simulink model "GHAME_Trim"  (R2024a)
settings: Solver=ode4  StartTime=0.0  StopTime=30  FixedStep=0.01  RelTol=1e-3
undefined symbols (not defined in the file): Data, IC, Sim
libraries: simulink_extras x4, sharedutil x2
settings Model: PauseTimes=399.98  PacingRate=1000  Creator=Thoma  LastModifiedBy=muel_td
settings SolverCC: AlgebraicLoopSolver=TrustRegion
settings DataIOCC: ExternalInput=getinputstruct(report2)  InitialState=getstatestruct(report2)
settings DebuggingCC: AlgebraicLoopMsg=none  InitInArrayFormatMsg=none  ArithmeticOperatorsInVariantConditions=warning
settings SFSimCC: CustomCodeUndefinedFunction=UseInterfaceOnly
settings RTWCC: GPUComputeCapability=3.5

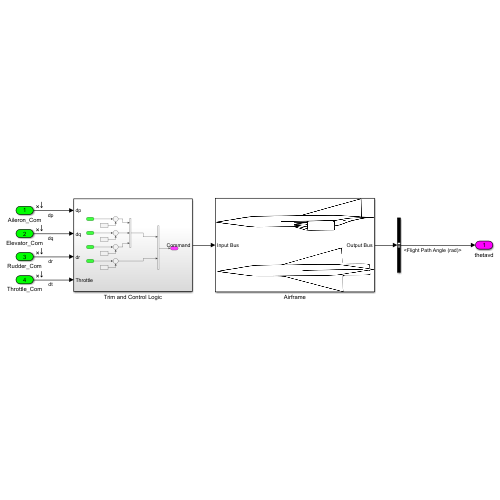
[thumbnail: Simulink's stored preview of the top-level diagram]
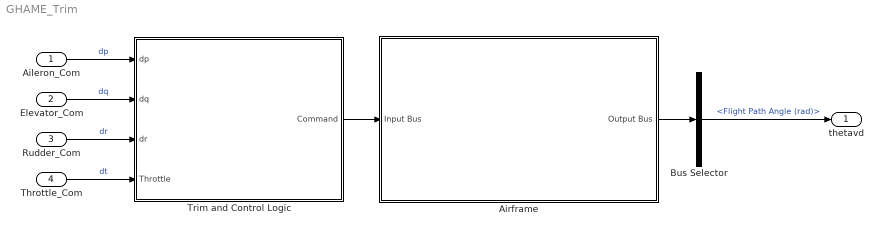
== system GHAME_Trim ==
  Aileron_Com : Inport  OutDataTypeStr=double
  Elevator_Com : Inport  Port=2  OutDataTypeStr=double
  Rudder_Com : Inport  Port=3  OutDataTypeStr=double
  Throttle_Com : Inport  Port=4
  Airframe : Subsystem
      mask Display: image('GHAME.png'); % Use "Edit Image" on toolstrip to change.
  Bus Selector : BusSelector  OutputSignals=Flight Path Angle (rad)
  Trim and Control Logic : Subsystem
  thetavd : Outport
  wires:
  Airframe/1(Output Bus) -> Bus Selector/1
  Bus Selector/1 -> thetavd/1  "<Flight Path Angle (rad)>"
  Aileron_Com/1 -> Trim and Control Logic/1(dp)  "dp"
  Elevator_Com/1 -> Trim and Control Logic/2(dq)  "dq"
  Rudder_Com/1 -> Trim and Control Logic/3(dr)  "dr"
  Throttle_Com/1 -> Trim and Control Logic/4(Throttle)  "dt"
  Trim and Control Logic/1(Command) -> Airframe/1(Input Bus)

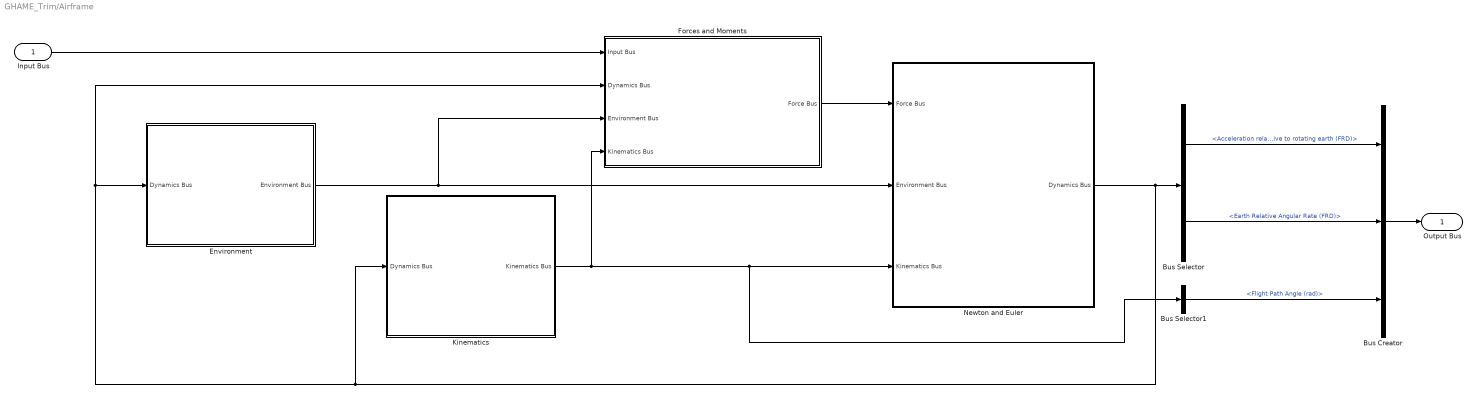
== system GHAME_Trim/Airframe ==
  Input Bus : Inport
  Bus Creator : BusCreator  Inputs=3
  Bus Selector : BusSelector  OutputSignals=Acceleration relative to rotating earth (FRD),Earth Relative Angular Rate (FRD)
  Bus Selector1 : BusSelector  OutputSignals=Flight Path Angle (rad)
  Environment : Subsystem
  Forces and Moments : Subsystem
  Kinematics : Subsystem
  Newton and Euler : Subsystem
  Output Bus : Outport
  wires:
  Newton and Euler/1(Dynamics Bus) -> Forces and Moments/2(Dynamics Bus), Environment/1(Dynamics Bus), Kinematics/1(Dynamics Bus), Bus Selector/1
  Kinematics/1(Kinematics Bus) -> Bus Selector1/1, Newton and Euler/3(Kinematics Bus), Forces and Moments/4(Kinematics Bus)
  Environment/1(Environment Bus) -> Forces and Moments/3(Environment Bus), Newton and Euler/2(Environment Bus)
  Forces and Moments/1(Force Bus) -> Newton and Euler/1(Force Bus)
  Input Bus/1 -> Forces and Moments/1(Input Bus)
  Bus Creator/1 -> Output Bus/1
  Bus Selector1/1 -> Bus Creator/3  "<Flight Path Angle (rad)>"
  Bus Selector/2 -> Bus Creator/2  "<Earth Relative Angular Rate (FRD)>"
  Bus Selector/1 -> Bus Creator/1  "<Acceleration relative to rotating earth (FRD)>"

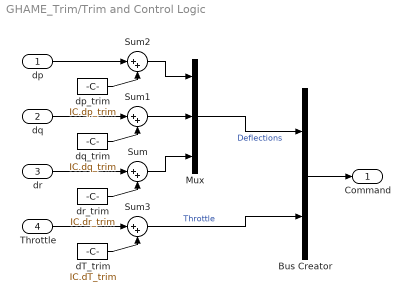
== system GHAME_Trim/Trim and Control Logic ==
  dp : Inport
  dq : Inport  Port=2
  dr : Inport  Port=3
  Throttle : Inport  Port=4
  Bus Creator : BusCreator  Inputs=2
  Mux : Mux  Inputs=3
  Sum{,1..3} (4 alike) : Sum  Inputs=|++
  dT_trim : Constant  Value=IC.dT_trim
  dp_trim : Constant  Value=IC.dp_trim
  dq_trim : Constant  Value=IC.dq_trim
  dr_trim : Constant  Value=IC.dr_trim
  Command : Outport
  wires:
  dr_trim/1 -> Sum/2
  Mux/1 -> Bus Creator/1  "Deflections"
  dq_trim/1 -> Sum1/2
  dp_trim/1 -> Sum2/2
  Sum/1 -> Mux/3
  Sum2/1 -> Mux/1
  Sum1/1 -> Mux/2
  dT_trim/1 -> Sum3/2
  Sum3/1 -> Bus Creator/2  "Throttle"
  Bus Creator/1 -> Command/1
  Throttle/1 -> Sum3/1
  dr/1 -> Sum/1
  dq/1 -> Sum1/1
  dp/1 -> Sum2/1

== system GHAME_Trim/Airframe/Environment ==
  Dynamics Bus : Inport
  Bus Creator : BusCreator  Inputs=5
  Bus Selector : BusSelector  OutputSignals=Geographic Velocity [NED],Geodetic Altitude,Inertial Position
  ENVIRONMENT : Subsystem
  Environment Bus : Outport
  wires:
  ENVIRONMENT/2(rho) -> Bus Creator/2  "Air Density"
  ENVIRONMENT/1(GRAVG) -> Bus Creator/1  "Gravitation (NED)"
  ENVIRONMENT/3(pdynmc) -> Bus Creator/3  "Dynamic Pressure"
  ENVIRONMENT/5(dvba) -> Bus Creator/5  "True Airspeed"
  ENVIRONMENT/4(vmach) -> Bus Creator/4  "Mach Number"
  Bus Creator/1 -> Environment Bus/1
  Dynamics Bus/1 -> Bus Selector/1
  Bus Selector/1 -> ENVIRONMENT/1(VBED)  "<Geographic Velocity [NED]>"
  Bus Selector/3 -> ENVIRONMENT/3(SBII)  "<Inertial Position>"
  Bus Selector/2 -> ENVIRONMENT/2(alt)  "<Geodetic Altitude>"

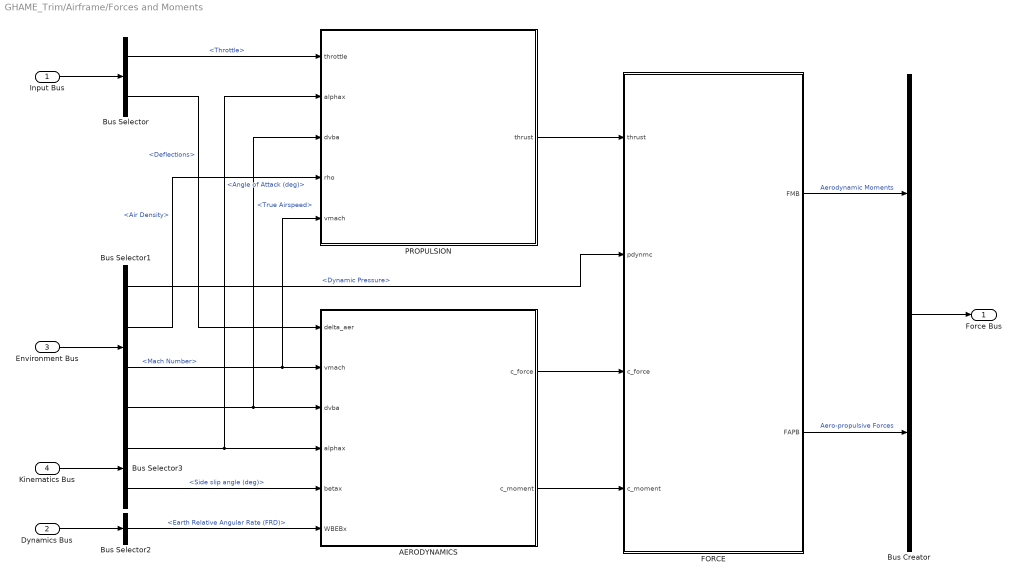
== system GHAME_Trim/Airframe/Forces and Moments ==
  Input Bus : Inport
  Dynamics Bus : Inport  Port=2
  Environment Bus : Inport  Port=3
  Kinematics Bus : Inport  Port=4
  AERODYNAMICS : Subsystem
  Bus Creator : BusCreator  Inputs=2
  Bus Selector : BusSelector  OutputSignals=Throttle,Deflections
  Bus Selector1 : BusSelector  OutputSignals=Dynamic Pressure,Air Density,Mach Number,True Airspeed
  Bus Selector2 : BusSelector  OutputSignals=Earth Relative Angular Rate (FRD)
  Bus Selector3 : BusSelector  OutputSignals=Angle of Attack (deg),Side slip angle (deg)
  FORCE : Subsystem
  PROPULSION : Subsystem
  Force Bus : Outport
  wires:
  Input Bus/1 -> Bus Selector/1
  Environment Bus/1 -> Bus Selector1/1
  Bus Selector/1 -> PROPULSION/1(throttle)  "<Throttle>"
  PROPULSION/1(thrust) -> FORCE/1(thrust)
  AERODYNAMICS/1(c_force) -> FORCE/3(c_force)
  AERODYNAMICS/2(c_moment) -> FORCE/4(c_moment)
  Bus Selector1/3 -> PROPULSION/5(vmach), AERODYNAMICS/2(vmach)  "<Mach Number>"
  Bus Selector1/4 -> PROPULSION/3(dvba), AERODYNAMICS/3(dvba)  "<True Airspeed>"
  Bus Selector1/2 -> PROPULSION/4(rho)  "<Air Density>"
  Dynamics Bus/1 -> Bus Selector2/1
  Bus Selector2/1 -> AERODYNAMICS/6(WBEBx)  "<Earth Relative Angular Rate (FRD)>"
  Kinematics Bus/1 -> Bus Selector3/1
  Bus Selector3/1 -> AERODYNAMICS/4(alphax), PROPULSION/2(alphax)  "<Angle of Attack (deg)>"
  Bus Selector3/2 -> AERODYNAMICS/5(betax)  "<Side slip angle (deg)>"
  FORCE/1(FMB) -> Bus Creator/1  "Aerodynamic Moments"
  FORCE/2(FAPB) -> Bus Creator/2  "Aero-propulsive Forces"
  Bus Creator/1 -> Force Bus/1
  Bus Selector/2 -> AERODYNAMICS/1(delta_aer)  "<Deflections>"
  Bus Selector1/1 -> FORCE/2(pdynmc)  "<Dynamic Pressure>"

== system GHAME_Trim/Airframe/Kinematics ==
  Dynamics Bus : Inport
  Bus Creator : BusCreator  Inputs=7
  Bus Selector : BusSelector  OutputSignals=Acceleration relative to rotating earth (FRD),Earth Relative Angular Rate (FRD),Geographic Velocity [NED],Inertial to Geodetic TM
  KINEMATICS : Subsystem
  Kinematics Bus : Outport
  wires:
  Dynamics Bus/1 -> Bus Selector/1
  Bus Selector/3 -> KINEMATICS/3(VBED)  "<Geographic Velocity [NED]>"
  Bus Selector/2 -> KINEMATICS/2(WBEBx)  "<Earth Relative Angular Rate (FRD)>"
  Bus Selector/1 -> KINEMATICS/1(a_BE_B)  "<Acceleration relative to rotating earth (FRD)>"
  KINEMATICS/1(e_BD) -> Bus Creator/1  "Euler Angles (rad)"
  KINEMATICS/2(TBD) -> Bus Creator/2  "Geodetic to Body TM"
  KINEMATICS/3(alphax) -> Bus Creator/3  "Angle of Attack (deg)"
  KINEMATICS/4(betax) -> Bus Creator/4  "Side slip angle (deg)"
  KINEMATICS/5(VBAB) -> Bus Creator/5  "Aerodynamic Velocity (FRD)"
  KINEMATICS/6(TBI) -> Bus Creator/6  "Inertial to Body TM"
  Bus Creator/1 -> Kinematics Bus/1
  Bus Selector/4 -> KINEMATICS/4(TDI)  "<Inertial to Geodetic TM>"
  KINEMATICS/7(thetavd) -> Bus Creator/7  "Flight Path Angle (rad)"

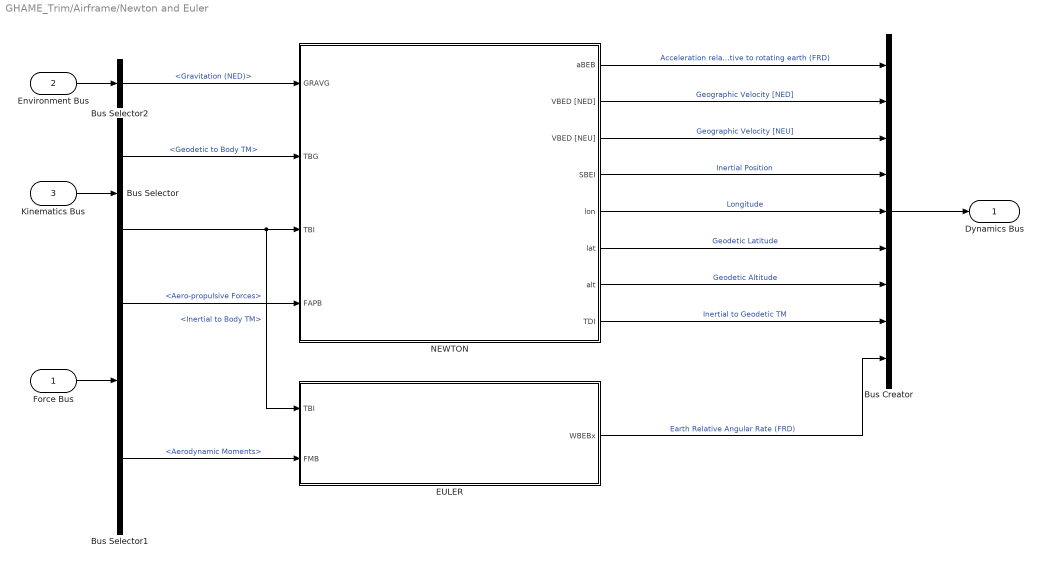
== system GHAME_Trim/Airframe/Newton and Euler ==
  Force Bus : Inport
  Environment Bus : Inport  Port=2
  Kinematics Bus : Inport  Port=3
  Bus Creator : BusCreator  Inputs=9
  Bus Selector : BusSelector  OutputSignals=Geodetic to Body TM,Inertial to Body TM
  Bus Selector1 : BusSelector  OutputSignals=Aero-propulsive Forces,Aerodynamic Moments
  Bus Selector2 : BusSelector  OutputSignals=Gravitation (NED)
  EULER : Subsystem
  NEWTON : Subsystem
  Dynamics Bus : Outport
  wires:
  Bus Selector1/2 -> EULER/2(FMB)  "<Aerodynamic Moments>"
  Bus Selector1/1 -> NEWTON/4(FAPB)  "<Aero-propulsive Forces>"
  Bus Creator/1 -> Dynamics Bus/1
  NEWTON/1(aBEB) -> Bus Creator/1  "Acceleration relative to rotating earth (FRD)"
  NEWTON/2(VBED [NED]) -> Bus Creator/2  "Geographic Velocity [NED]"
  NEWTON/3(VBED [NEU]) -> Bus Creator/3  "Geographic Velocity [NEU]"
  NEWTON/4("SBEI ") -> Bus Creator/4  "Inertial Position"
  NEWTON/5(lon) -> Bus Creator/5  "Longitude"
  NEWTON/6(lat) -> Bus Creator/6  "Geodetic Latitude"
  NEWTON/7(alt) -> Bus Creator/7  "Geodetic Altitude"
  Kinematics Bus/1 -> Bus Selector/1
  Bus Selector/2 -> NEWTON/3(TBI), EULER/1(TBI)  "<Inertial to Body TM>"
  Force Bus/1 -> Bus Selector1/1
  Bus Selector/1 -> NEWTON/2(TBG)  "<Geodetic to Body TM>"
  Environment Bus/1 -> Bus Selector2/1
  Bus Selector2/1 -> NEWTON/1(GRAVG)  "<Gravitation (NED)>"
  NEWTON/8(TDI) -> Bus Creator/8  "Inertial to Geodetic TM"
  EULER/1(WBEBx) -> Bus Creator/9  "Earth Relative Angular Rate (FRD)"

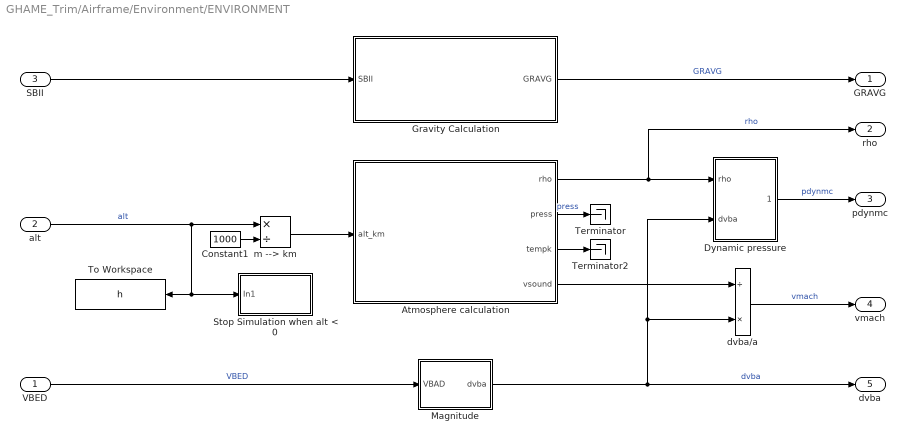
== system GHAME_Trim/Airframe/Environment/ENVIRONMENT ==
  VBED : Inport
  alt : Inport  Port=2
  SBII : Inport  Port=3
  Atmosphere calculation : MATLAB Function  Priority=2  TreatAsAtomicUnit=on
  Constant1 : Constant  Value=1000
  Dynamic pressure : Subsystem
  Gravity Calculation : MATLAB Function  Priority=1  TreatAsAtomicUnit=on
  Magnitude : MATLAB Function  TreatAsAtomicUnit=on
  Stop Simulation when alt < 0 : Subsystem
  Terminator : Terminator
  Terminator2 : Terminator
  To Workspace : ToWorkspace  VariableName=h  SampleTime=-1
  dvba/a : Product  Inputs=/*
  m --> km : Product  Inputs=*/
  GRAVG : Outport
  rho : Outport  Port=2
  pdynmc : Outport  Port=3
  vmach : Outport  Port=4
  dvba : Outport  Port=5
  wires:
  alt/1 -> To Workspace/1, Stop Simulation when alt < 0/1(In1), m --> km/1  "alt"
  Atmosphere calculation/3(tempk) -> Terminator2/1
  Constant1/1 -> m --> km/2
  m --> km/1 -> Atmosphere calculation/1(alt_km)
  dvba/a/1 -> vmach/1  "vmach"
  Atmosphere calculation/1(rho) -> Dynamic pressure/1(rho), rho/1  "rho"
  Dynamic pressure/1(pdynmc) -> pdynmc/1  "pdynmc"
  Atmosphere calculation/4(vsound) -> dvba/a/1
  Magnitude/1(dvba) -> dvba/a/2, Dynamic pressure/2(dvba), dvba/1  "dvba"
  Gravity Calculation/1(GRAVG) -> GRAVG/1  "GRAVG"
  SBII/1 -> Gravity Calculation/1(SBII)
  VBED/1 -> Magnitude/1(VBAD)  "VBED"
  Atmosphere calculation/2(press) -> Terminator/1  "press"

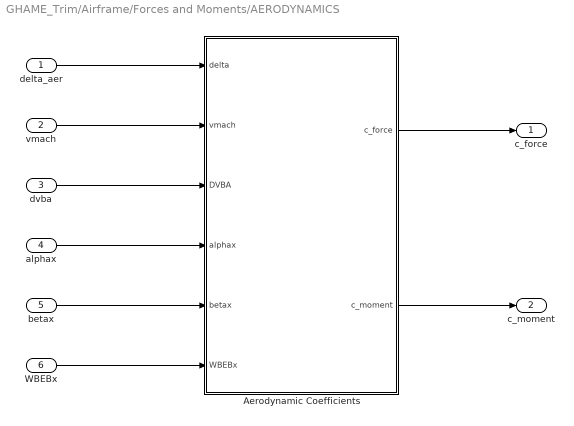
== system GHAME_Trim/Airframe/Forces and Moments/AERODYNAMICS ==
  delta_aer : Inport
  vmach : Inport  Port=2
  dvba : Inport  Port=3
  alphax : Inport  Port=4
  betax : Inport  Port=5
  WBEBx : Inport  Port=6
  Aerodynamic Coefficients : MATLAB Function  TreatAsAtomicUnit=on
  c_force : Outport  PortDimensions=[3 1]
  c_moment : Outport  Port=2  PortDimensions=[3 1]
  wires:
  vmach/1 -> Aerodynamic Coefficients/2(vmach)
  dvba/1 -> Aerodynamic Coefficients/3(DVBA)
  betax/1 -> Aerodynamic Coefficients/5(betax)
  alphax/1 -> Aerodynamic Coefficients/4(alphax)
  Aerodynamic Coefficients/1(c_force) -> c_force/1
  WBEBx/1 -> Aerodynamic Coefficients/6(WBEBx)
  Aerodynamic Coefficients/2(c_moment) -> c_moment/1
  delta_aer/1 -> Aerodynamic Coefficients/1(delta)

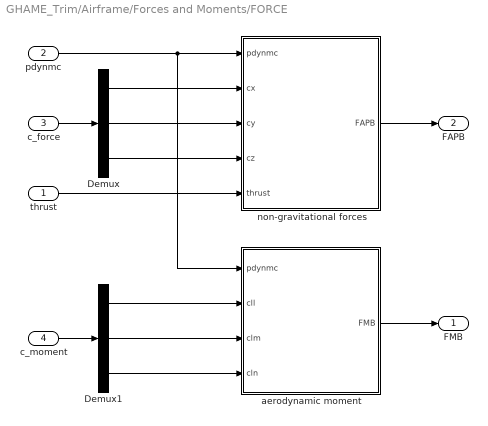
== system GHAME_Trim/Airframe/Forces and Moments/FORCE ==
  thrust : Inport
  pdynmc : Inport  Port=2
  c_force : Inport  Port=3  PortDimensions=[3 1]
  c_moment : Inport  Port=4  PortDimensions=[3 1]
  Demux : Demux  Outputs=3
  Demux1 : Demux  Outputs=3
  aerodynamic moment : MATLAB Function  TreatAsAtomicUnit=on
  non-gravitational forces : MATLAB Function  TreatAsAtomicUnit=on
  FMB : Outport
  FAPB : Outport  Port=2
  wires:
  Demux/1 -> non-gravitational forces/2(cx)
  c_force/1 -> Demux/1
  Demux/3 -> non-gravitational forces/4(cz)
  non-gravitational forces/1(FAPB) -> FAPB/1
  Demux1/1 -> aerodynamic moment/2(cll)
  c_moment/1 -> Demux1/1
  Demux1/3 -> aerodynamic moment/4(cln)
  aerodynamic moment/1(FMB) -> FMB/1
  Demux/2 -> non-gravitational forces/3(cy)
  Demux1/2 -> aerodynamic moment/3(clm)
  thrust/1 -> non-gravitational forces/5(thrust)
  pdynmc/1 -> non-gravitational forces/1(pdynmc), aerodynamic moment/1(pdynmc)

== system GHAME_Trim/Airframe/Forces and Moments/PROPULSION ==
  throttle : Inport
  alphax : Inport  Port=2
  dvba : Inport  Port=3
  rho : Inport  Port=4
  vmach : Inport  Port=5
  making thrust calculations : MATLAB Function  TreatAsAtomicUnit=on
  thrust : Outport
  wires:
  rho/1 -> making thrust calculations/1(rho)
  dvba/1 -> making thrust calculations/4(DVBA)
  vmach/1 -> making thrust calculations/2(Mach)
  making thrust calculations/1(Thrust) -> thrust/1  "Thrust"
  alphax/1 -> making thrust calculations/3(alphax)
  throttle/1 -> making thrust calculations/5(Throttle)

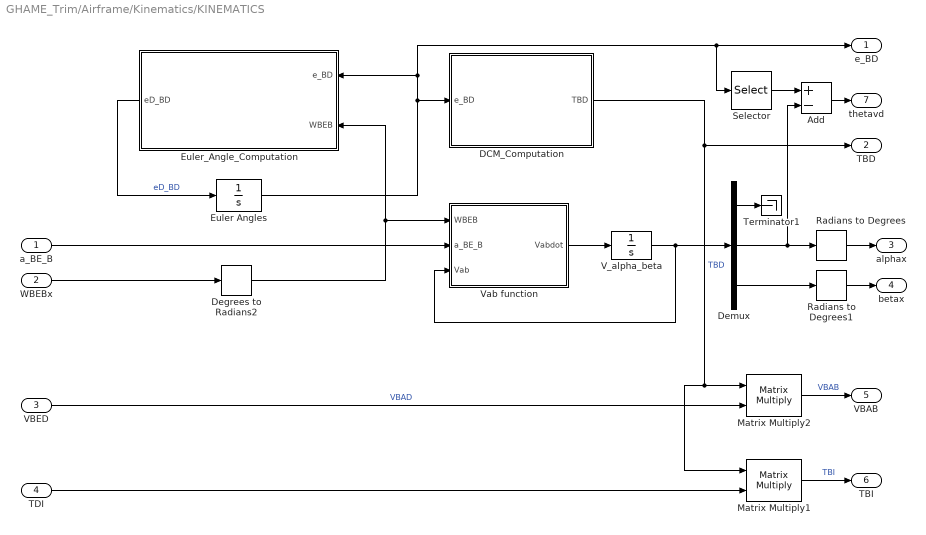
== system GHAME_Trim/Airframe/Kinematics/KINEMATICS ==
  a_BE_B : Inport
  WBEBx : Inport  Port=2
  VBED : Inport  Port=3
  TDI : Inport  Port=4
  Add : Sum  Inputs=+-
  DCM_Computation : MATLAB Function  TreatAsAtomicUnit=on
  Degrees to Radians2 : simulink_extras/Transformations/Degrees to Radians
  Demux : Demux  Outputs=3
  Euler Angles : Integrator  InitialCondition=[IC.psibd; IC.thtbd; IC.phibd]
  Euler_Angle_Computation : MATLAB Function  TreatAsAtomicUnit=on
  Matrix Multiply1 : Product  Multiplication=Matrix(*)
  Matrix Multiply2 : Product  Multiplication=Matrix(*)
  Radians to Degrees : simulink_extras/Transformations/Radians to Degrees
  Radians to Degrees1 : simulink_extras/Transformations/Radians to Degrees
  Selector : Selector  InputPortWidth=3  IndexOptions=Index vector (dialog)  Indices=[2]  OutputSizes=1
  Terminator1 : Terminator
  V_alpha_beta : Integrator  InitialCondition=[IC.dvba; IC.alpha; 0]
  Vab function : MATLAB Function  TreatAsAtomicUnit=on
  e_BD : Outport
  TBD : Outport  Port=2
  alphax : Outport  Port=3
  betax : Outport  Port=4
  VBAB : Outport  Port=5
  TBI : Outport  Port=6
  thetavd : Outport  Port=7
  wires:
  Matrix Multiply1/1 -> TBI/1  "TBI"
  VBED/1 -> Matrix Multiply2/2  "VBAD"
  WBEBx/1 -> Degrees to Radians2/1
  Euler Angles/1 -> e_BD/1, Selector/1, Euler_Angle_Computation/1(e_BD), DCM_Computation/1(e_BD)
  DCM_Computation/1(TBD) -> TBD/1, Matrix Multiply1/1, Matrix Multiply2/1  "TBD"
  Euler_Angle_Computation/1(eD_BD) -> Euler Angles/1  "eD_BD"
  Vab function/1(Vabdot) -> V_alpha_beta/1
  V_alpha_beta/1 -> Vab function/3(Vab), Demux/1
  Demux/1 -> Terminator1/1
  Demux/3 -> Radians to Degrees1/1
  a_BE_B/1 -> Vab function/2(a_BE_B)
  Degrees to Radians2/1 -> Euler_Angle_Computation/2(WBEB), Vab function/1(WBEB)
  Demux/2 -> Radians to Degrees/1, Add/2
  Matrix Multiply2/1 -> VBAB/1  "VBAB"
  TDI/1 -> Matrix Multiply1/2
  Selector/1 -> Add/1
  Add/1 -> thetavd/1
  Radians to Degrees/1 -> alphax/1
  Radians to Degrees1/1 -> betax/1

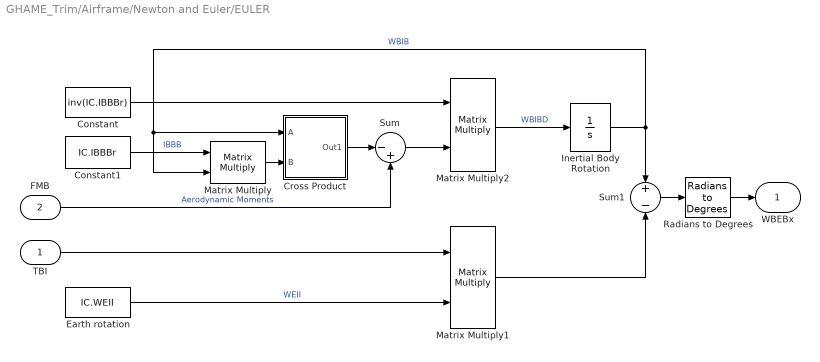
== system GHAME_Trim/Airframe/Newton and Euler/EULER ==
  TBI : Inport
  FMB : Inport  Port=2
  Constant : Constant  Value=inv(IC.IBBBr)
  Constant1 : Constant  Value=IC.IBBBr
  Cross Product : Subsystem
  Earth rotation : Constant  Value=IC.WEII
  Inertial Body Rotation : Integrator  InitialCondition=IC.WBIB
  Matrix Multiply : Product  Multiplication=Matrix(*)
  Matrix Multiply1 : Product  Multiplication=Matrix(*)
  Matrix Multiply2 : Product  Multiplication=Matrix(*)
  Radians to Degrees : simulink_extras/Transformations/Radians to Degrees
  Sum : Sum  Inputs=|-+
  Sum1 : Sum  Inputs=+-
  WBEBx : Outport
  wires:
  FMB/1 -> Sum/2  "Aerodynamic Moments"
  Matrix Multiply2/1 -> Inertial Body Rotation/1  "WBIBD"
  Constant1/1 -> Matrix Multiply/1  "IBBB"
  Inertial Body Rotation/1 -> Sum1/1, Cross Product/1(A), Matrix Multiply/2  "WBIB"
  Matrix Multiply/1 -> Cross Product/2(B)
  Sum/1 -> Matrix Multiply2/2
  Radians to Degrees/1 -> WBEBx/1
  Cross Product/1(Out1) -> Sum/1
  Constant/1 -> Matrix Multiply2/1
  TBI/1 -> Matrix Multiply1/1
  Earth rotation/1 -> Matrix Multiply1/2  "WEII"
  Matrix Multiply1/1 -> Sum1/2
  Sum1/1 -> Radians to Degrees/1

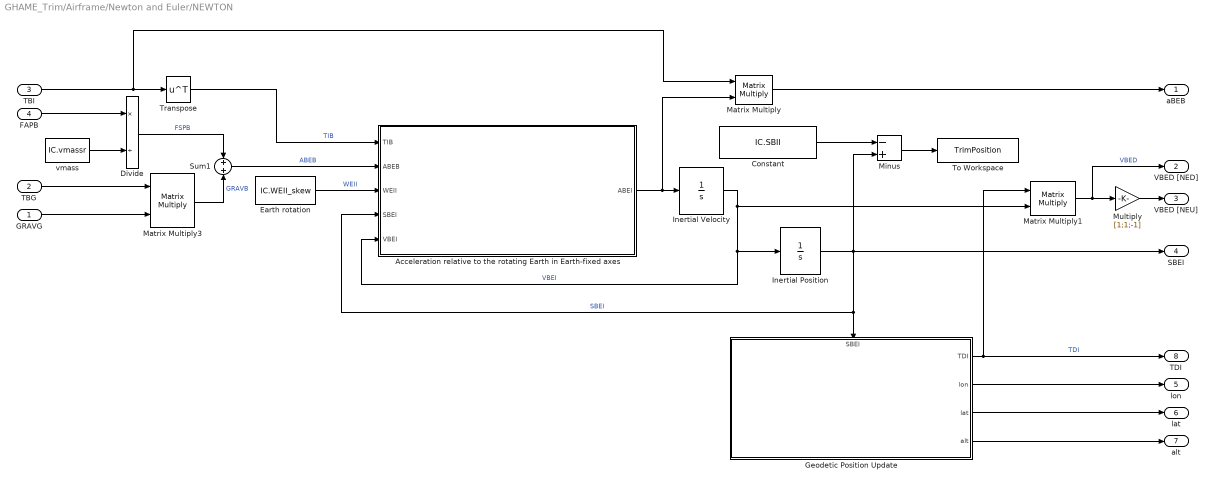
== system GHAME_Trim/Airframe/Newton and Euler/NEWTON ==
  GRAVG : Inport
  TBG : Inport  Port=2
  TBI : Inport  Port=3
  FAPB : Inport  Port=4
  Acceleration relative to the rotating Earth in Earth-fixed axes : Subsystem
  Constant : Constant  Value=IC.SBII  SampleTime=Sim.sample_time
  Divide : Product  Inputs=*/
  Earth rotation : Constant  Value=IC.WEII_skew
  Geodetic Position Update : Subsystem
      settings: PortSchema="{\"entries\":[{\"content\":{\"sides\":[{\"content\":{},\"type\":\"ConnectorPlacement.EquallySpacedRectSide\",\"uuid\":\"95933ad7-71e7-41f9-a46f-bd289a95730a\"},{\"content\":{\"connectorIds\":[\"Out1\",\"Out2\",\"Out3\",\"Out4\"],\"side\":\"RIGHT\"},\"type\":\"ConnectorPlacement.EquallySpacedRectSide\",\"uuid\":\"ab2689fc-78b4-4a63-be7d-36d19ac80c5e\"},{\"content\":{\"connectorIds\":[\"In1\"],\"side\":\"TOP\"},\"type\":\"ConnectorPlacement.EquallySpacedRectSide\",\"uuid\":\"1c090c4e-beeb-4e17-b6f2-47983e28fdde\"}]},\"type\":\"ConnectorPlacement.EquallySpacedConnector\",\"uuid\":\"92176c65-9b1a-45aa-814d-7bd7a5ccaffc\"}],\"packageUris\":[\"http://schema.mathworks.com/mf0/Connector/R2020b\"],\"version\":\"1.0\"}"
  Inertial Position : Integrator  InitialCondition=IC.SBII
  Inertial Velocity : Integrator  InitialCondition=IC.VBEI
  Matrix Multiply : Product  Multiplication=Matrix(*)
  Matrix Multiply1 : Product  Multiplication=Matrix(*)
  Matrix Multiply3 : Product  Multiplication=Matrix(*)
  Minus : Sum  Inputs=-+
  Multiply : Gain  Gain=[1;1;-1]
  Sum1 : Sum
  To Workspace : ToWorkspace  VariableName=TrimPosition  SaveFormat=Timeseries  SampleTime=-1
  Transpose : Math  Operator=transpose  SignedPower=on
  vmass : Constant  Value=IC.vmassr
  aBEB : Outport
  VBED [NED] : Outport  Port=2
  VBED [NEU] : Outport  Port=3
  "SBEI " : Outport  Port=4
  lon : Outport  Port=5
  lat : Outport  Port=6
  alt : Outport  Port=7
  TDI : Outport  Port=8
  wires:
  TBG/1 -> Matrix Multiply3/1
  GRAVG/1 -> Matrix Multiply3/2
  Divide/1 -> Sum1/1  "FSPB"
  vmass/1 -> Divide/2
  Matrix Multiply1/1 -> VBED [NED]/1, Multiply/1  "VBED"
  FAPB/1 -> Divide/1
  Matrix Multiply3/1 -> Sum1/2  "GRAVB"
  Multiply/1 -> VBED [NEU]/1
  Inertial Velocity/1 -> Acceleration relative to the rotating Earth in Earth-fixed axes/5(VBEI), Inertial Position/1, Matrix Multiply1/2  "VBEI"
  Inertial Position/1 -> "SBEI "/1, Minus/2, Geodetic Position Update/1(SBEI), Acceleration relative to the rotating Earth in Earth-fixed axes/4(SBEI)  "SBEI"
  TBI/1 -> Matrix Multiply/1, Transpose/1
  Geodetic Position Update/1(TDI) -> TDI/1, Matrix Multiply1/1  "TDI"
  Geodetic Position Update/4(alt) -> alt/1
  Geodetic Position Update/3(lat) -> lat/1
  Geodetic Position Update/2(lon) -> lon/1
  Constant/1 -> Minus/1
  Minus/1 -> To Workspace/1
  Matrix Multiply/1 -> aBEB/1
  Acceleration relative to the rotating Earth in Earth-fixed axes/1(ABEI) -> Matrix Multiply/2, Inertial Velocity/1
  Transpose/1 -> Acceleration relative to the rotating Earth in Earth-fixed axes/1(TIB)  "TIB"
  Sum1/1 -> Acceleration relative to the rotating Earth in Earth-fixed axes/2(ABEB)  "ABEB"
  Earth rotation/1 -> Acceleration relative to the rotating Earth in Earth-fixed axes/3(WEII)  "WEII"

== system GHAME_Trim/Airframe/Environment/ENVIRONMENT/Dynamic pressure ==
  rho : Inport
  dvba : Inport  Port=2
  Gain : Gain  Gain=0.5
  Product : Product
  Square : Math  Operator=square  SignedPower=on
  pdynmc : Outport
  wires:
  Gain/1 -> pdynmc/1
  Product/1 -> Gain/1
  rho/1 -> Product/2
  dvba/1 -> Square/1
  Square/1 -> Product/1

== system GHAME_Trim/Airframe/Environment/ENVIRONMENT/Stop Simulation when alt < 0 ==
  In1 : Inport
  If : If  IfExpression=u1 <= 25  ShowElse=off
  Stop Simulationalt<0 : Subsystem  TreatAsAtomicUnit=on
  wires:
  If/1 -> Stop Simulationalt<0/Action
  In1/1 -> If/1

== system GHAME_Trim/Airframe/Newton and Euler/EULER/Cross Product ==
  A : Inport
  B : Inport  Port=2
  Subsystem : sharedutil/3x3 Cross Product/Subsystem  SystemSampleTime=-1  VariantActivationTime=update diagram  AllowFlexibleInterface=on  Latency=0  AutoFrameSizeCalculation=off
  Subsystem1 : sharedutil/3x3 Cross Product/Subsystem1  SystemSampleTime=-1  VariantActivationTime=update diagram  AllowFlexibleInterface=on  Latency=0  AutoFrameSizeCalculation=off
  Sum : Sum  Inputs=+|-  InputSameDT=on  SaturateOnIntegerOverflow=on  OutDataTypeStr=Inherit: Same as first input
  Out1 : Outport
  wires:
  Subsystem/1 -> Sum/1
  B/1 -> Subsystem/2, Subsystem1/2
  A/1 -> Subsystem1/1, Subsystem/1
  Subsystem1/1 -> Sum/2
  Sum/1 -> Out1/1

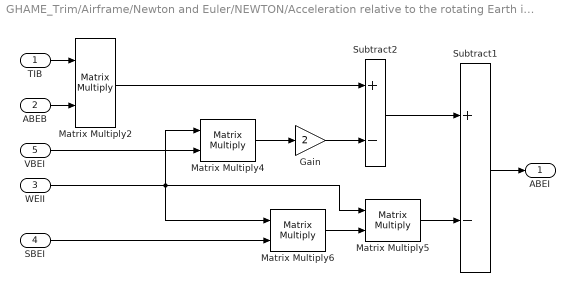
== system GHAME_Trim/Airframe/Newton and Euler/NEWTON/Acceleration relative to the rotating Earth in Earth-fixed axes ==
  TIB : Inport
  ABEB : Inport  Port=2
  WEII : Inport  Port=3
  SBEI : Inport  Port=4
  VBEI : Inport  Port=5
  Gain : Gain  Gain=2
  Matrix Multiply{2,4..6} (4 alike) : Product  Multiplication=Matrix(*)
  Subtract1 : Sum  Inputs=+-
  Subtract2 : Sum  Inputs=+-
  ABEI : Outport
  wires:
  Gain/1 -> Subtract2/2
  Matrix Multiply4/1 -> Gain/1
  Subtract2/1 -> Subtract1/1
  SBEI/1 -> Matrix Multiply6/2
  Matrix Multiply2/1 -> Subtract2/1
  VBEI/1 -> Matrix Multiply4/2
  WEII/1 -> Matrix Multiply6/1, Matrix Multiply4/1, Matrix Multiply5/1
  Matrix Multiply6/1 -> Matrix Multiply5/2
  Matrix Multiply5/1 -> Subtract1/2
  ABEB/1 -> Matrix Multiply2/2
  TIB/1 -> Matrix Multiply2/1
  Subtract1/1 -> ABEI/1

== system GHAME_Trim/Airframe/Newton and Euler/NEWTON/Geodetic Position Update ==
  SBEI : Inport
  Find Geodetic Position : MATLAB Function  TreatAsAtomicUnit=on
  Inertial to Geodetic : MATLAB Function  TreatAsAtomicUnit=on
  TDI : Outport
  lon : Outport  Port=2
  lat : Outport  Port=3
  alt : Outport  Port=4
  wires:
  SBEI/1 -> Find Geodetic Position/1(SBII)
  Find Geodetic Position/1(lon) -> Inertial to Geodetic/1("lon ")
  Find Geodetic Position/2(lat) -> Inertial to Geodetic/2("lat ")
  Find Geodetic Position/3(alt) -> Inertial to Geodetic/3("alt ")
  Inertial to Geodetic/1(TDI) -> TDI/1  "TDI"
  Inertial to Geodetic/4(alt) -> alt/1
  Inertial to Geodetic/3(lon) -> lon/1
  Inertial to Geodetic/2(lat) -> lat/1

== system GHAME_Trim/Airframe/Environment/ENVIRONMENT/Stop Simulation when alt < 0/Stop Simulationalt<0 ==
  Action Port : ActionPort  ActionPortLabel=if(u1 <= 25)
  Constant2 : Constant
  Stop Simulation : Stop
  wires:
  Constant2/1 -> Stop Simulation/1

== matlab function GHAME_Trim/Airframe/Environment/ENVIRONMENT/Gravity Calculation ==
  data: SBII input; GRAVG output; Sim parameter
function GRAVG = cad_grav84(SBII, Sim)
% CAD_GRAV84  Gravitational acceleration of the WGS-84 Earth including the
%   J2 term, in geocentric local-level axes.
%
%   GRAVG = cad_grav84(SBII, Sim)
%
%   Gradient of the potential
%     U = GM/r * (1 + sqrt(5)*C20*(a/r)^2 * (3*sin(latc)^2 - 1)/2)
%   with the normalized second zonal harmonic C20 (negative for the oblate
%   Earth). The field is rotationally symmetric about the polar axis, so it
%   depends only on the distance and the geocentric latitude, not on
%   longitude or time. The east component is zero. C20 = 0 gives the
%   point-mass field of the spherical Earth model.
%
%   Inputs
%     SBII   [3x1]  Position in inertial (or Earth-fixed) axes (m)
%     Sim    struct Earth constants Sim.earth.GM, SMAJOR_AXIS, C20
%
%   Output
%     GRAVG  [3x1]  Gravitational acceleration [north; east; down] in
%                   geocentric local-level axes (m/s^2)

%   Author:    Thomas Harald Müller
%   GitHub:    https://github.com/ThomasHaraldMueller
%   Copyright: (c) 2026 Thomas Harald Müller, Hamburg, Germany
%   Free to use and modify, provided this notice is kept and the author is credited.

GM  = Sim.earth.GM;
a   = Sim.earth.SMAJOR_AXIS;
C20 = Sim.earth.C20;

% Distance and geocentric latitude
dbi  = norm(SBII);
slat = SBII(3) / dbi;               % sin(latc)
clat = sqrt(1 - slat^2);            % cos(latc) >= 0

% Common factors
g0 = GM / dbi^2;                    % Point-mass gravity
k  = sqrt(5) * C20 * (a / dbi)^2;   % J2 scaling

GRAVG = [ 3 * g0 * k * slat * clat;               % North, towards the equator for C20 < 0
          0;                                      % East
          g0 * (1 + 1.5 * k * (3 * slat^2 - 1)) ];% Down

end

== matlab function GHAME_Trim/Airframe/Kinematics/KINEMATICS/DCM_Computation ==
  data: TBD output; e_BD input
function TBD = DCM_Computation(e_BD)
% DCM_COMPUTATION  Direction cosine matrix of the body relative to the
%   local-level frame from the 3-2-1 Euler angles.
%
%   TBD = DCM_Computation(e_BD)
%
%   Built analytically from the angles, so it is orthogonal to machine
%   precision
%
%   Input
%     e_BD  [3x1]  Euler angles [phi; theta; psi] (rad)
%
%   Output
%     TBD   [3x3]  Transformation from local-level to body axes

%   Author:    Thomas Harald Müller
%   GitHub:    https://github.com/ThomasHaraldMueller
%   Copyright: (c) 2026 Thomas Harald Müller, Hamburg, Germany
%   Free to use and modify, provided this notice is kept and the author is credited.

sphi = sin(e_BD(1));   cphi = cos(e_BD(1));
stht = sin(e_BD(2));   ctht = cos(e_BD(2));
spsi = sin(e_BD(3));   cpsi = cos(e_BD(3));

TBD = [ cpsi*ctht,                    spsi*ctht,                    -stht;
        cpsi*stht*sphi - spsi*cphi,   spsi*stht*sphi + cpsi*cphi,   ctht*sphi;
        cpsi*stht*cphi + spsi*sphi,   spsi*stht*cphi - cpsi*sphi,   ctht*cphi ];

end

== matlab function GHAME_Trim/Airframe/Kinematics/KINEMATICS/Euler_Angle_Computation ==
  data: e_BD input; WBEB input; eD_BD output
function eD_BD = Euler_Angle_Computation(e_BD, WBEB)
% EULER_ANGLE_COMPUTATION  Euler angle rates of the body relative to the
%   local-level frame for the 3-2-1 sequence (yaw, pitch, roll).
%
%   eD_BD = Euler_Angle_Computation(e_BD, WBEB)
%
%   Uses the body rate relative to the Earth. The rotation of the local-level
%   frame over the Earth (about V/R) is neglected. Singular at theta = +-90 deg.
%
%   Inputs
%     e_BD   [3x1]  Euler angles [phi; theta; psi] (rad)
%     WBEB   [3x1]  Body rate relative to the Earth in body axes [p; q; r] (rad/s)
%
%   Output
%     eD_BD  [3x1]  Euler angle rates [phi_dot; theta_dot; psi_dot] (rad/s)

%   Author:    Thomas Harald Müller
%   GitHub:    https://github.com/ThomasHaraldMueller
%   Copyright: (c) 2026 Thomas Harald Müller, Hamburg, Germany
%   Free to use and modify, provided this notice is kept and the author is credited.

sphi = sin(e_BD(1));
cphi = cos(e_BD(1));
ctht = cos(e_BD(2));
ttht = tan(e_BD(2));

q = WBEB(2);
r = WBEB(3);

% Pitch and yaw components of the rate in the roll plane
q_r_sin = q * sphi + r * cphi;

eD_BD = [ WBEB(1) + q_r_sin * ttht;
          q * cphi - r * sphi;
          q_r_sin / ctht ];

end

== matlab function GHAME_Trim/Airframe/Kinematics/KINEMATICS/Vab function ==
  data: WBEB input; a_BE_B input; Vab input; Vabdot output
function Vabdot = Vab_Dynamics(WBEB, a_BE_B, Vab)
% VAB_DYNAMICS  Rates of speed, angle of attack and sideslip relative to
%   the Earth.
%
%   Vabdot = Vab_Dynamics(WBEB, a_BE_B, Vab)
%
%   Follows from d/dt|B v = d/dt|E v - WBEB x v with the body velocity
%   v = V [cos(alpha)cos(beta); sin(beta); sin(alpha)cos(beta)].
%   The acceleration must be taken relative to the rotating Earth, i.e.
%   a_BE_B = TBI * ABEI including the Coriolis and centrifugal terms.
%   Singular at V = 0 and beta = +-90 deg.
%
%   Inputs
%     WBEB    [3x1]  Body rate relative to the Earth in body axes [p; q; r] (rad/s)
%     a_BE_B  [3x1]  Acceleration relative to the Earth in body axes (m/s^2)
%     Vab     [3x1]  [V (m/s); alpha (rad); beta (rad)]
%
%   Output
%     Vabdot  [3x1]  [V_dot (m/s^2); alpha_dot (rad/s); beta_dot (rad/s)]

%   Author:    Thomas Harald Müller
%   GitHub:    https://github.com/ThomasHaraldMueller
%   Copyright: (c) 2026 Thomas Harald Müller, Hamburg, Germany
%   Free to use and modify, provided this notice is kept and the author is credited.

V = Vab(1);
salp = sin(Vab(2));   calp = cos(Vab(2));
sbet = sin(Vab(3));   cbet = cos(Vab(3));

p = WBEB(1);   q = WBEB(2);   r = WBEB(3);
ax = a_BE_B(1);   ay = a_BE_B(2);   az = a_BE_B(3);

% Acceleration along the velocity and normal to it in the symmetry plane
a_par  = calp*ax + salp*az;
a_norm = calp*az - salp*ax;

Vabdot = [ cbet*a_par + sbet*ay;
           q - (p*calp + r*salp)*sbet/cbet + a_norm/(V*cbet);
           p*salp - r*calp + (cbet*ay - sbet*a_par)/V ];

end

== matlab function GHAME_Trim/Airframe/Forces and Moments/AERODYNAMICS/Aerodynamic Coefficients ==
  data: delta input; c_force output double size=[3 1]; vmach input; DVBA input; alphax input; betax input; WBEBx input; c_moment output double size=[3 1]; Data parameter; Sim parameter
function [c_force, c_moment] = aerodynamics(delta, vmach, DVBA, alphax, betax, WBEBx, Data, Sim)
% AERODYNAMICS  Aerodynamic force and moment coefficients of the GHAME
%   vehicle from the tabulated aero database.
%
%   [c_force, c_moment] = aerodynamics(delta, vmach, DVBA, alphax, betax, ...
%       WBEBx, Data, Sim)
%
%   Used in the plant. For Monte Carlo runs pass UNC.Perturbed from
%   Create_Uncertainty as Data, otherwise the nominal Data. The tables are
%   interpolated bilinearly in Mach and alpha, clamped to the table range.
%
%   Inputs
%     delta   [3x1]  Control surface deflections [aileron, elevator, rudder] (rad)
%     vmach   [1x1]  Mach number
%     DVBA    [1x1]  Airspeed (m/s)
%     alphax  [1x1]  Angle of attack (deg)
%     betax   [1x1]  Sideslip angle (deg)
%     WBEBx   [3x1]  Body rates [p, q, r] (deg/s)
%     Data    struct Aero tables and breakpoints (Data.AeroCoefficients)
%     Sim     struct Constants and vehicle geometry
%
%   Outputs
%     c_force   [3x1]  Body-axis force coefficients [Cx, Cy, Cz]
%     c_moment  [3x1]  Body-axis moment coefficients [Cl, Cm, Cn]
%
%   All table derivatives are per degree.

%   Author:    Thomas Harald Müller
%   GitHub:    https://github.com/ThomasHaraldMueller
%   Copyright: (c) 2026 Thomas Harald Müller, Hamburg, Germany
%   Free to use and modify, provided this notice is kept and the author is credited.

%% Constants and geometry
RAD  = Sim.constants.RAD;
DEG  = Sim.constants.DEG;
refb = Sim.vehicle.geometry.refb;
refc = Sim.vehicle.geometry.refc;

% Deflections in table units (deg)
delax = delta(1) * DEG;
delex = delta(2) * DEG;
delrx = delta(3) * DEG;

ppx = WBEBx(1);
qqx = WBEBx(2);
rrx = WBEBx(3);

%% Table lookup
Aero      = Data.AeroCoefficients;
alpha_vec = Aero.alpha_vec;             % Breakpoints from the database (deg)
mach_vec  = Aero.Mach_vec;

vmach_c  = clamp_value(vmach,  mach_vec(1),  mach_vec(end));
alphax_c = clamp_value(alphax, alpha_vec(1), alpha_vec(end));

interp_coeff = @(table) interp2(mach_vec, alpha_vec, table, vmach_c, alphax_c, 'linear');

%% Stability-axis force coefficients
% Drag
cd0 = interp_coeff(Aero.CD0_tab);
cda = interp_coeff(Aero.CDA_tab);
cd  = cd0 + cda * alphax;

% Lift
cl0  = interp_coeff(Aero.CL0_tab);
cla  = interp_coeff(Aero.CLA_tab);
clde = interp_coeff(Aero.CLDE_tab);
cl   = cl0 + cla * alphax + clde * delex;

% Side force
cyb  = interp_coeff(Aero.CYB_tab);
cyda = interp_coeff(Aero.CYDA_tab);
cydr = interp_coeff(Aero.CYDR_tab);
cy   = cyb * betax + cyda * delax + cydr * delrx;

%% Body-axis moment coefficients
% Rate damping terms use the nondimensional rates p*b/(2V), q*c/(2V), r*b/(2V)
pn = ppx * RAD * refb / (2 * DVBA);
qn = qqx * RAD * refc / (2 * DVBA);
rn = rrx * RAD * refb / (2 * DVBA);

% Rolling moment
cllb  = interp_coeff(Aero.CLLB_tab);
cllda = interp_coeff(Aero.CLLDA_tab);
clldr = interp_coeff(Aero.CLLDR_tab);
cllp  = interp_coeff(Aero.CLLP_tab);
cllr  = interp_coeff(Aero.CLLR_tab);
cll   = cllb * betax + cllda * delax + clldr * delrx + cllp * pn + cllr * rn;

% Pitching moment
cm0  = interp_coeff(Aero.CM0_tab);
cma  = interp_coeff(Aero.CMA_tab);
cmde = interp_coeff(Aero.CMDE_tab);
cmq  = interp_coeff(Aero.CMQ_tab);
clm  = cm0 + cma * alphax + cmde * delex + cmq * qn;

% Yawing moment
clnb  = interp_coeff(Aero.CNB_tab);
clnda = interp_coeff(Aero.CNDA_tab);
clndr = interp_coeff(Aero.CNDR_tab);
clnp  = interp_coeff(Aero.CNP_tab);
clnr  = interp_coeff(Aero.CNR_tab);
cln   = clnb * betax + clnda * delax + clndr * delrx + clnp * pn + clnr * rn;

%% Body-axis outputs
% Rotation from stability axes (CD, CL) to body axes (Cx, Cz)
a  = alphax * RAD;
Cx = -cd * cos(a) + cl * sin(a);
Cz = -cd * sin(a) - cl * cos(a);

c_force  = [Cx; cy; Cz];
c_moment = [cll; clm; cln];

end

%% Local functions

function value_clamped = clamp_value(value, min_value, max_value)
% CLAMP_VALUE  Saturate value to [min_value, max_value]
    value_clamped = max(min(value, max_value), min_value);
end

== matlab function GHAME_Trim/Airframe/Forces and Moments/FORCE/aerodynamic moment ==
  data: pdynmc input; FMB output; cll input; clm input; cln input; Sim parameter
function FMB = computeMoment(pdynmc, cll, clm, cln, Sim)
% COMPUTEMOMENT  Aerodynamic moments in body axes from the moment coefficients.
%
%   FMB = computeMoment(pdynmc, cll, clm, cln, Sim)
%
%   Roll and yaw are referenced to the span, pitch to the chord. Thrust acts
%   along the body x-axis through the centre of gravity and adds no moment.
%
%   Inputs
%     pdynmc  [1x1]  Dynamic pressure (Pa)
%     cll     [1x1]  Rolling moment coefficient
%     clm     [1x1]  Pitching moment coefficient
%     cln     [1x1]  Yawing moment coefficient
%     Sim     struct Reference geometry (refa, refb, refc)
%
%   Output
%     FMB     [3x1]  Aerodynamic moments [L; M; N] in body axes (N m)

%   Author:    Thomas Harald Müller
%   GitHub:    https://github.com/ThomasHaraldMueller
%   Copyright: (c) 2026 Thomas Harald Müller, Hamburg, Germany
%   Free to use and modify, provided this notice is kept and the author is credited.

qS   = pdynmc * Sim.vehicle.geometry.refa;
refb = Sim.vehicle.geometry.refb;
refc = Sim.vehicle.geometry.refc;

FMB = qS * [refb * cll;
            refc * clm;
            refb * cln];

end

== matlab function GHAME_Trim/Airframe/Forces and Moments/FORCE/non-gravitational forces ==
  data: pdynmc input; FAPB output size=[3 1]; cx input; cy input; cz input; thrust input; Sim parameter
function FAPB = computeForces(pdynmc, cx, cy, cz, thrust, Sim)
% COMPUTEFORCES  Aerodynamic and propulsive forces in body axes.
%
%   FAPB = computeForces(pdynmc, cx, cy, cz, thrust, Sim)
%
%   Sum of the aerodynamic forces and the thrust, which acts along the body
%   x-axis. Gravity is not included. Divided by the mass this gives the
%   specific force FSPB.
%
%   Inputs
%     pdynmc  [1x1]  Dynamic pressure (Pa)
%     cx      [1x1]  Axial force coefficient in body axes
%     cy      [1x1]  Side force coefficient in body axes
%     cz      [1x1]  Normal force coefficient in body axes
%     thrust  [1x1]  Thrust along the body x-axis (N)
%     Sim     struct Reference geometry (refa)
%
%   Output
%     FAPB    [3x1]  Aerodynamic and propulsive forces in body axes (N)

%   Author:    Thomas Harald Müller
%   GitHub:    https://github.com/ThomasHaraldMueller
%   Copyright: (c) 2026 Thomas Harald Müller, Hamburg, Germany
%   Free to use and modify, provided this notice is kept and the author is credited.

qS = pdynmc * Sim.vehicle.geometry.refa;

FAPB = qS * [cx; cy; cz] + [thrust; 0; 0];

end

== matlab function GHAME_Trim/Airframe/Forces and Moments/PROPULSION/making thrust calculations ==
  data: rho input; Mach input; alphax input; DVBA input; Data parameter; Throttle input; Thrust output; Sim parameter
function Thrust = Thrust_Computation(rho, Mach, alphax, DVBA, Data, Throttle, Sim)
% THRUST_COMPUTATION  Scramjet thrust for the trim model.
%
%   Thrust = Thrust_Computation(rho, Mach, alphax, DVBA, Data, Throttle, Sim)
%
%   Same engine model as thrust.m, reduced to the thrust. The engine is
%   modelled through the captured air mass flow
%
%     mdot_air  = rho * V * A_capture * acowl
%     mdot_fuel = FAR_ST * Throttle * mdot_air
%     Thrust    = Isp(Mach, Throttle) * g0 * mdot_fuel
%
%   Mach, alpha and throttle are clamped to the table range.
%
%   Inputs
%     rho       [1x1]  Atmospheric density (kg/m^3)
%     Mach      [1x1]  Mach number
%     alphax    [1x1]  Angle of attack (deg)
%     DVBA      [1x1]  Airspeed (m/s)
%     Data      struct Engine tables (Data.ThrustCoefficients)
%     Throttle  [1x1]  Commanded equivalence ratio
%     Sim       struct Constants and vehicle geometry
%
%   Output
%     Thrust    [1x1]  Thrust along the body x-axis (N)

%   Author:    Thomas Harald Müller
%   GitHub:    https://github.com/ThomasHaraldMueller
%   Copyright: (c) 2026 Thomas Harald Müller, Hamburg, Germany
%   Free to use and modify, provided this notice is kept and the author is credited.

%% Constants
thrtl_idle = 0.05;      % Minimum equivalence ratio
thrtl_max  = 2;         % Maximum equivalence ratio
FAR_ST     = 0.029;     % Stoichiometric fuel-air ratio (hydrogen)

AGRAV = Sim.earth.AGRAV;
acowl = Sim.vehicle.acowl;

%% Engine tables
Mach_vec     = Data.ThrustCoefficients.Mach_vec;
alpha_vec    = Data.ThrustCoefficients.alpha_vec;       % deg
throttle_vec = Data.ThrustCoefficients.throttle_vec;

capture_area_tab = Data.ThrustCoefficients.Capture_A;   % f(Mach, alpha)
SPI_tab          = Data.ThrustCoefficients.SPI_tab;     % f(Mach, Throttle), s

%% Table lookups
Throttle = max(min(Throttle, thrtl_max), thrtl_idle);

% Clamp to the table range so that interp2 cannot return NaN
Mach_c  = max(min(Mach,     Mach_vec(end)),     Mach_vec(1));
alpha_c = max(min(alphax,   alpha_vec(end)),    alpha_vec(1));
thr_c   = max(min(Throttle, throttle_vec(end)), throttle_vec(1));

SPI          = interp2(Mach_vec, throttle_vec, SPI_tab,          Mach_c, thr_c,   'linear');
capture_area = interp2(Mach_vec, alpha_vec,    capture_area_tab, Mach_c, alpha_c, 'linear');

%% Thrust
mdot_air  = rho * DVBA * capture_area * acowl;
mdot_fuel = FAR_ST * Throttle * mdot_air;

Thrust = SPI * AGRAV * mdot_fuel;

end

== matlab function GHAME_Trim/Airframe/Environment/ENVIRONMENT/Magnitude ==
  data: VBAD input; dvba output
function dvba = fcn(VBAD)

dvba = sqrt(VBAD(1)^2+VBAD(2)^2+VBAD(3)^2);

== matlab function GHAME_Trim/Airframe/Newton and Euler/NEWTON/Geodetic Position Update/Find Geodetic Position ==
  data: SBII input; lon output; Sim parameter; lat output; alt output
function [lon, lat, alt] = cad_geo84_in_cont(SBII, Sim)
% CAD_GEO84_IN_CONT  Inertial position to geodetic longitude, latitude and
%   altitude on the WGS-84 ellipsoid, at the initial epoch.
%
%   [lon, lat, alt] = cad_geo84_in_cont(SBII, Sim)
%
%   Trim version for the initial epoch t = 0. The Earth has not rotated yet,
%   so the angle WEII3*t vanishes and the celestial longitude equals
%   GW_CLONG plus the geodetic longitude. Earth rotation itself is still
%   part of the trim model. Latitude and altitude use Bowring's closed-form
%   method, accurate to well below a millimetre for altitudes up to orbital
%   heights.
%
%   Inputs
%     SBII   [3x1]  Position in inertial coordinates (m)
%     Sim    struct Ellipsoid parameters (flattening, semi-major axis) and
%                   Greenwich longitude at the initial epoch (rad)
%
%   Outputs
%     lon    [1x1]  Geodetic longitude in (-pi, pi] (rad)
%     lat    [1x1]  Geodetic latitude (rad)
%     alt    [1x1]  Altitude above the ellipsoid (m)

%   Author:    Thomas Harald Müller
%   GitHub:    https://github.com/ThomasHaraldMueller
%   Copyright: (c) 2026 Thomas Harald Müller, Hamburg, Germany
%   Free to use and modify, provided this notice is kept and the author is credited.

%% Ellipsoid
f = Sim.earth.FLATTENING;
a = Sim.earth.SMAJOR_AXIS;

b   = a * (1 - f);              % Semi-minor axis
e2  = 2*f - f^2;                % First eccentricity squared
ep2 = e2 / (1 - e2);            % Second eccentricity squared

x = SBII(1);
y = SBII(2);
z = SBII(3);

%% Longitude
% Rotation angle WEII3*t is zero at the initial epoch
lon = atan2(y, x) - Sim.earth.GW_CLONG;
lon = atan2(sin(lon), cos(lon));                 % Wrap to (-pi, pi]

%% Latitude (Bowring)
p = sqrt(x^2 + y^2);                            % Distance from the polar axis
u = atan2(z * a, p * b);                        % Parametric latitude

lat = atan2(z + ep2 * b * sin(u)^3, ...
            p - e2  * a * cos(u)^3);

%% Altitude
% Form valid at all latitudes, including the poles
N   = a / sqrt(1 - e2 * sin(lat)^2);            % Prime vertical radius of curvature
alt = p * cos(lat) + z * sin(lat) - a^2 / N;

end

== matlab function GHAME_Trim/Airframe/Newton and Euler/NEWTON/Geodetic Position Update/Inertial to Geodetic ==
  data: lon input; TDI output; lat output; lon output; lat input; alt input; Sim parameter; alt output
function [TDI, lat, lon, alt] = cad_tdi84(lon, lat, alt, Sim)
% CAD_TDI84  Transformation matrix from inertial to geodetic coordinates
%   at the initial epoch.
%
%   [TDI, lat, lon, alt] = cad_tdi84(lon, lat, alt, Sim)
%
%   Trim version for t = 0. The rotation angle WEII3*t is zero at the initial
%   epoch, so the celestial longitude equals GW_CLONG plus the geodetic
%   longitude.
%   The geodetic frame D is north, east, down at the vehicle position.
%
%   Inputs
%     lon   [1x1]  Geodetic longitude (rad)
%     lat   [1x1]  Geodetic latitude (rad)
%     alt   [1x1]  Altitude above the ellipsoid (m)
%     Sim   struct Greenwich longitude at the initial epoch (rad)
%
%   Outputs
%     TDI   [3x3]  Transformation matrix, v_D = TDI * v_I
%     lat, lon, alt  Passed through unchanged

%   Author:    Thomas Harald Müller
%   GitHub:    https://github.com/ThomasHaraldMueller
%   Copyright: (c) 2026 Thomas Harald Müller, Hamburg, Germany
%   Free to use and modify, provided this notice is kept and the author is credited.

% Celestial longitude
lon_cel = Sim.earth.GW_CLONG + lon;

slat = sin(lat);
clat = cos(lat);
slon = sin(lon_cel);
clon = cos(lon_cel);

TDI = [ -slat*clon,  -slat*slon,   clat;     % North
        -slon,        clon,        0;        % East
        -clat*clon,  -clat*slon,  -slat ];   % Down

end

== matlab function GHAME_Trim/Airframe/Environment/ENVIRONMENT/Atmosphere calculation ==
  data: rho output; press output; tempk output; vsound output; alt_km input
function [rho, press, tempk, vsound] = us76_nasa2002(alt_km)
% US76_NASA2002  1976 U.S. Standard Atmosphere from 0 to 1000 km.
%
%   [rho, press, tempk, vsound] = us76_nasa2002(alt_km)
%
%   Below 86 km the standard layers with linear temperature in geopotential
%   altitude are evaluated analytically. Above 86 km temperature follows the
%   standard piecewise model, while pressure and molecular weight are
%   interpolated quadratically (pressure in log scale) between table points.
%   Altitudes outside [0, 1000] km are clamped to the range.
%
%   Input
%     alt_km  [1x1]  Geometric altitude (km)
%
%   Outputs
%     rho     [1x1]  Density (kg/m^3)
%     press   [1x1]  Pressure (Pa)
%     tempk   [1x1]  Temperature (K)
%     vsound  [1x1]  Speed of sound (m/s), with gamma = 1.4

%   Author:    Thomas Harald Müller
%   GitHub:    https://github.com/ThomasHaraldMueller
%   Copyright: (c) 2026 Thomas Harald Müller, Hamburg, Germany
%   Free to use and modify, provided this notice is kept and the author is credited.

%% Constants
ro  = 6356.766;     % Effective Earth radius for geopotential altitude (km)
go  = 9.80665;      % Standard gravity (m/s^2)
wmo = 28.9644;      % Sea-level molecular weight (kg/kmol)
rs  = 8314.32;      % Universal gas constant (J/(kmol K))

%% Tables
% Altitude breakpoints (km)
zs = [0, 11.019, 20.063, 32.162, 47.35, 51.413, 71.802, 86, 91, 94, ...
      97, 100, 103, 106, 108, 110, 112, 115, 120, 125, 130, 135, 140, ...
      145, 150, 155, 160, 165, 170, 180, 190, 210, 230, 265, 300, 350, ...
      400, 450, 500, 550, 600, 650, 700, 750, 800, 850, 900, 950, 1000];

% Temperature (K)
tms = [288.15, 216.65, 216.65, 228.65, 270.65, 270.65, 214.65, ...
       186.95, 186.87, 187.74, 190.40, 195.08, 202.23, 212.89, ...
       223.29, 240.00, 264.00, 300.00, 360.00, 417.23, 469.27, ...
       516.59, 559.63, 598.78, 634.39, 666.80, 696.29, 723.13, ...
       747.57, 790.07, 825.31, 878.84, 915.78, 955.20, 976.01, ...
       990.06, 995.83, 998.22, 999.24, 999.67, 999.85, 999.93, ...
       999.97, 999.99, 999.99, 1000, 1000, 1000, 1000];

% Molecular weight (kg/kmol)
wms = [28.9644, 28.9644, 28.9644, 28.9644, 28.9644, 28.9644, ...
       28.9644, 28.9522, 28.8890, 28.7830, 28.6200, 28.3950, ...
       28.1040, 27.7650, 27.5210, 27.2680, 27.0200, 26.6800, ...
       26.2050, 25.8030, 25.4360, 25.0870, 24.7490, 24.4220, ...
       24.1030, 23.7920, 23.4880, 23.1920, 22.9020, 22.3420, ...
       21.8090, 20.8250, 19.9520, 18.6880, 17.7260, 16.7350, ...
       15.9840, 15.2470, 14.3300, 13.0920, 11.5050, 9.7180, ...
       7.9980, 6.5790, 5.5430, 4.8490, 4.4040, 4.1220, 3.9400];

% Pressure (tabulated in hPa, converted to Pa)
ps = [1013.25, 226.32, 54.7487, 8.68014, 1.10905, 0.66938, ...
      0.039564, 3.7338e-03, 1.5381e-03, 9.0560e-04, 5.3571e-04, ...
      3.2011e-04, 1.9742e-04, 1.2454e-04, 9.3188e-05, 7.1042e-05, ...
      5.5547e-05, 4.0096e-05, 2.5382e-05, 1.7354e-05, 1.2505e-05, ...
      9.3568e-06, 7.2028e-06, 5.6691e-06, 4.5422e-06, 3.6930e-06, ...
      3.0395e-06, 2.5278e-06, 2.1210e-06, 1.5271e-06, 1.1266e-06, ...
      6.4756e-07, 3.9276e-07, 1.7874e-07, 8.7704e-08, 3.4498e-08, ...
      1.4518e-08, 6.4468e-09, 3.0236e-09, 1.5137e-09, 8.2130e-10, ...
      4.8865e-10, 3.1908e-10, 2.2599e-10, 1.7036e-10, 1.3415e-10, ...
      1.0873e-10, 8.9816e-11, 7.5138e-11] * 100;

%% Layer index
alt_km = min(max(alt_km, 0), 1000);
n = numel(zs);

% Interval i with zs(i) <= alt_km < zs(i+1), limited to the last interval.
% A plain loop keeps i a fixed-size scalar for code generation.
i = 1;
while i < n - 1 && zs(i+1) <= alt_km
    i = i + 1;
end

%% Layers 1 to 7 (0 to 86 km), analytic in geopotential altitude
if i <= 7
    zl = ro * zs(i)   / (ro + zs(i));       % Geopotential altitudes (km)
    zu = ro * zs(i+1) / (ro + zs(i+1));
    ht = ro * alt_km  / (ro + alt_km);

    lapse = (tms(i+1) - tms(i)) / (zu - zl);   % Temperature gradient (K/km)
    tempk = tms(i) + lapse * (ht - zl);
    wm    = wmo;

    if abs(lapse) > 1e-12
        press = ps(i) * (tms(i) / tempk)^(go * wmo / (rs * lapse * 1e-3));
    else
        press = ps(i) * exp(-go * wmo * (ht - zl) * 1e3 / (rs * tms(i)));
    end

%% Layers above 86 km, standard temperature model and table interpolation
else
    if i == 8                       % 86 to 91 km, isothermal at 186.87 K
        tempk = tms(9);
    elseif i <= 15                  % 91 to 110 km, elliptical
        tempk = 263.1905 - 76.3232 * sqrt(1 - ((alt_km - 91) / 19.9429)^2);
    elseif i <= 18                  % 110 to 120 km, linear
        tempk = 240 + 12 * (alt_km - 110);
    else                            % Above 120 km, exponential
        xi    = (alt_km - 120) * (ro + 120) / (ro + alt_km);
        tempk = 1000 - 640 * exp(-0.01875 * xi);
    end

    % Quadratic interpolation over the interval and its upper neighbour
    j = i;
    if i == n - 1
        j = i - 1;                  % Keep the stencil inside the table
    end
    [wma, lpa] = lagrange3(zs, wms, log(ps), j, alt_km);
    wmb = wma;
    lpb = lpa;

    % Average with the stencil shifted one point down, except at the ends
    if i ~= 8 && i ~= n - 1
        [wmb, lpb] = lagrange3(zs, wms, log(ps), j - 1, alt_km);
    end

    press = exp((lpa + lpb) / 2);
    wm    = (wma + wmb) / 2;
end

%% Density and speed of sound
rho    = wm * press / (rs * tempk);
vsound = sqrt(1.4 * press / rho);

end

%% Local functions

function [y1, y2] = lagrange3(z, f1, f2, j, x)
% LAGRANGE3  Quadratic Lagrange interpolation of two tables through the
%   points j, j+1 and j+2.
    z0 = z(j);  z1 = z(j+1);  z2 = z(j+2);
    L0 = (x - z1) * (x - z2) / ((z0 - z1) * (z0 - z2));
    L1 = (x - z0) * (x - z2) / ((z1 - z0) * (z1 - z2));
    L2 = (x - z0) * (x - z1) / ((z2 - z0) * (z2 - z1));
    y1 = f1(j) * L0 + f1(j+1) * L1 + f1(j+2) * L2;
    y2 = f2(j) * L0 + f2(j+1) * L1 + f2(j+2) * L2;
end
